simulink model "mySimulink"  (R2020a)
settings: Solver=VariableStepAuto  StartTime=0.0  StopTime=0.5  RelTol=1e-3
values from neighbouring files (symbols this model uses):
  Cr1_t = Cr0    (= 0.001)    [TPMCC.m]
  Cr2_t = Cr0    (= 0.001)    [TPMCC.m]
  f = 10^-6    (= 1e-06)    [TPMCC.m]
  Jm = 9.19*10^-7    (= 9.19e-07)    [TPMCC.m]
  Kc = 1.63*10^-2    (= 0.0163)    [TPMCC.m]
  Ke = 30/pi*585    (= 5586.33850253)    [TPMCC.m]
  Komega = pi*1.75/(30*10^3)    (= 0.000183259571459)    [TPMCC.m]
  L = 0.12*10^-4    (= 1.2e-05)    [TPMCC.m]
  R = 1.34    [TPMCC.m]
  Rc = 0    [TPMCC.m]
  Rtilde = R    (= 1.34)    [TPMCC.m]
  x = 36    [TPMCC.m]
settings Model: Creator=gaetan  LastModifiedBy=gaetan

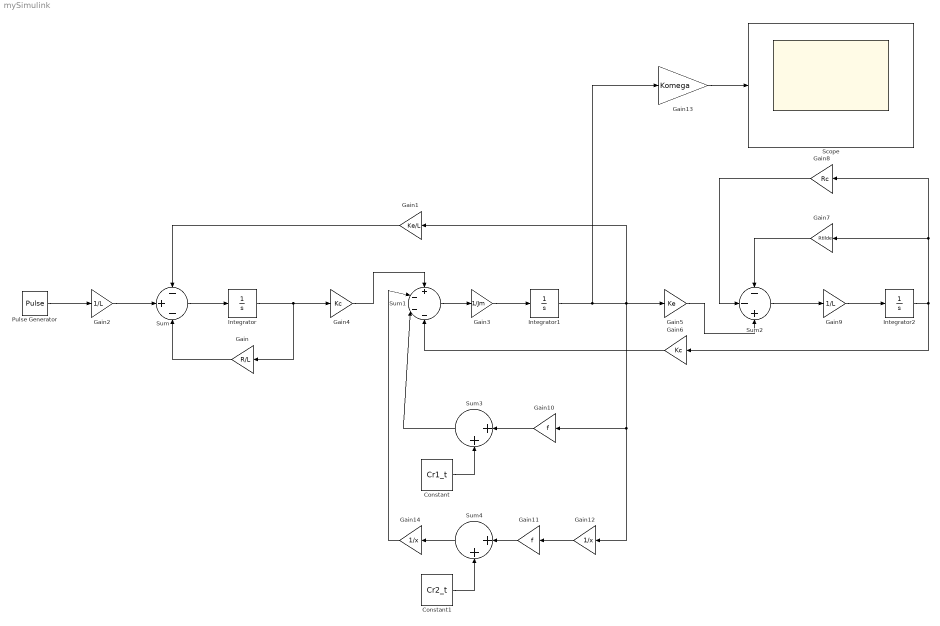
== system mySimulink ==
  Constant : Constant  Value=Cr1_t
  Constant1 : Constant  Value=Cr2_t
  Gain : Gain  Gain=R/L
  Gain1 : Gain  Gain=Ke/L
  Gain10 : Gain  Gain=f
  Gain11 : Gain  Gain=f
  Gain12 : Gain  Gain=1/x
  Gain13 : Gain  Gain=Komega
  Gain14 : Gain  Gain=1/x
  Gain2 : Gain  Gain=1/L
  Gain3 : Gain  Gain=1/Jm
  Gain4 : Gain  Gain=Kc
  Gain5 : Gain  Gain=Ke
  Gain6 : Gain  Gain=Kc
  Gain7 : Gain  Gain=Rtilde
  Gain8 : Gain  Gain=Rc
  Gain9 : Gain  Gain=1/L
  Integrator : Integrator
  Integrator1 : Integrator
  Integrator2 : Integrator
  Pulse Generator : DiscretePulseGenerator  PulseType=Time based  Amplitude=10  Period=0.1  PulseWidth=50
  Scope : Scope
  Sum : Sum  Inputs=-+-
  Sum1 : Sum  Inputs=+---
  Sum2 : Sum  Inputs=--+
  Sum3 : Sum  Inputs=|++
  Sum4 : Sum  Inputs=|++
  wires:
  Sum/1 -> Integrator/1
  Gain2/1 -> Sum/2
  Integrator1/1 -> Gain13/1, Gain12/1, Gain10/1, Gain5/1, Gain1/1
  Integrator/1 -> Gain4/1, Gain/1
  Pulse Generator/1 -> Gain2/1
  Gain1/1 -> Sum/1
  Gain/1 -> Sum/3
  Gain4/1 -> Sum1/1
  Sum1/1 -> Gain3/1
  Gain3/1 -> Integrator1/1
  Gain6/1 -> Sum1/4
  Gain5/1 -> Sum2/3
  Gain7/1 -> Sum2/1
  Gain8/1 -> Sum2/2
  Sum2/1 -> Gain9/1
  Gain9/1 -> Integrator2/1
  Integrator2/1 -> Gain8/1, Gain7/1, Gain6/1
  Sum3/1 -> Sum1/3
  Sum4/1 -> Gain14/1
  Gain10/1 -> Sum3/1
  Gain11/1 -> Sum4/1
  Constant/1 -> Sum3/2
  Constant1/1 -> Sum4/2
  Gain12/1 -> Gain11/1
  Gain13/1 -> Scope/1
  Gain14/1 -> Sum1/2
